simulink model "flightControlSystem"  (R2026a)
settings: Solver=ode3  StartTime=0  StopTime=TFinal  FixedStep=Ts  EnableMultiTasking=on
undefined symbols (not defined in the file): codertarget, Controller, DiscIntNeverNeededParam, Discrete, Estimator, g, init, Sensors, Time, Ts, var_acc_angle_N, var_bias_gyr_N, var_gyro_p_N, Vehicle
libraries: simulink x39, slpidlib x4, ctrlSharedLib x4, sharedtransform x3, parrotlib x1
(part 1 of 2)
settings Model: ExtModeTrigDuration=80  Creator=The MathWorks, Inc.  LastModifiedBy=The MathWorks, Inc.
settings DataIOCC: SaveFormat=StructureWithTime
settings OptimizationCC: PassReuseOutputArgsThreshold=0.0
settings DebuggingCC: ParameterPrecisionLossMsg=none  BusObjectLabelMismatch=error  PregeneratedLibrarySubsystemCodeDiagnostic=none
settings HardwareCC: ProdLargestAtomicInteger=Long  ProdHWDeviceType=ARM Compatible->ARM 9  UseEmbeddedCoderFeatures=off  UseSimulinkCoderFeatures=off
settings ModelReferenceCC: ModelReferenceNumInstancesAllowed=Single
settings RTWCC: SystemTargetFile=ert.tlc  HardwareBoard=PARROT Mambo  TLCOptions=-aInlineSetEventsForThisBaseRateFcn=TLC_FALSE -aSuppressMultiTaskScheduler=TLC_FALSE -aRateBasedStepFcn=1  Toolchain=Sourcery G++ Lite GNU Toolchain for Drones  Description=Embedded Coder
settings CodeAppCC: MaxIdLength=63.0
settings ERTTargetCC: ExtModeMaxTrigDuration=80.0  DynamicArrayContainerType=coder::array  ERTCustomFileBanners=off  MatFileLogging=on  SubcomponentCodeInterfacePackaging=Nonreusable function  SupportContinuousTime=on  SupportNonInlinedSFcns=on  ModelStepFunctionPrototypeControlCompliant=off
settings SimscapeCC: SimscapeLogType=none  SimscapeNominalValues="[{\"value\":\"1\",\"unit\":\"A\"},{\"value\":\"1\",\"unit\":\"bar\"},{\"value\":\"1\",\"unit\":\"cm^2\"},{\"value\":\"1\",\"unit\":\"cm^3/s\"},{\"value\":\"1\",\"unit\":\"kJ/kg\"},{\"value\":\"1\",\"unit\":\"kW\"},{\"value\":\"1\",\"unit\":\"l\"},{\"value\":\"1\",\"unit\":\"N\"},{\"value\":\"1\",\"unit\":\"N*m\"},{\"value\":\"1\",\"unit\":\"V\"}]"  SimscapeLogDataHistory=5000  SimscapeLogDecimation=1

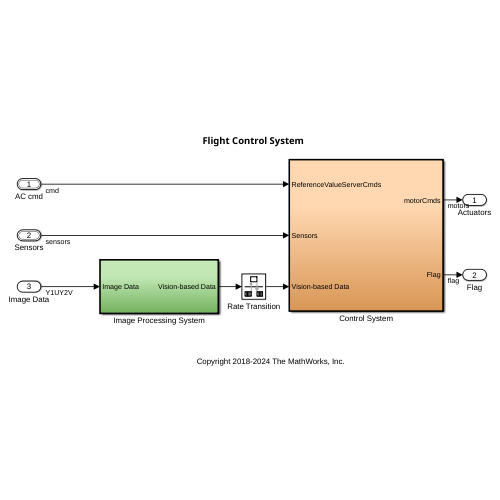
[thumbnail: Simulink's stored preview of the top-level diagram]
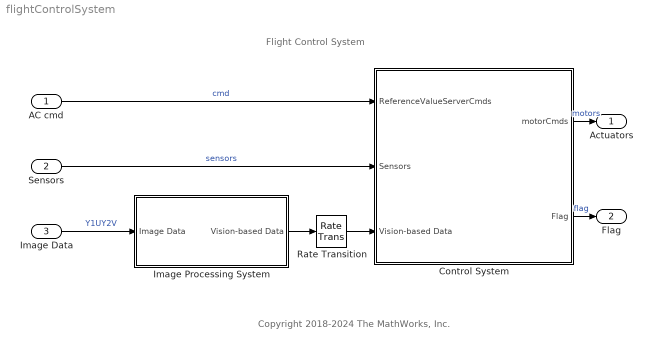
== system flightControlSystem ==
  note: Copyright 2018-2024 The MathWorks, Inc.
  note: Flight Control System
  AC cmd : Inport  OutDataTypeStr=Bus: CommandBus  BusOutputAsStruct=on
  Sensors : Inport  Port=2  OutDataTypeStr=Bus: SensorsBus  BusOutputAsStruct=on
  Image Data : Inport  Tag=IP_IN  InitFcn=codertarget.parrot.internal.inportCallback(gcb);  Port=3  OutDataTypeStr=uint8  PortDimensions=[4 9600]  BusOutputAsStruct=on
  Control System : Subsystem  InitFcn=codertarget.parrot.internal.fcsSubsystemCallback(gcb);  TreatAsAtomicUnit=on  SystemSampleTime=Ts
  Image Processing System : Subsystem  Tag=IP_SUB  InitFcn=codertarget.parrot.internal.ipSubsystemCallback(gcb);  TreatAsAtomicUnit=on  SystemSampleTime=40*Ts  RTWFcnName=ImageFunction
      settings: RTWSystemCode=Inline  RTWFcnNameOpts=User specified
  Rate Transition : RateTransition  Deterministic=off
  Actuators : Outport  OutDataTypeStr=single  PortDimensions=4  VectorParamsAs1DForOutWhenUnconnected=off
  Flag : Outport  Port=2  OutDataTypeStr=uint8  PortDimensions=1  VectorParamsAs1DForOutWhenUnconnected=off
  wires:
  AC cmd/1 -> Control System/1(ReferenceValueServerCmds)  "cmd"
  Control System/1(motorCmds) -> Actuators/1  "motors"
  Sensors/1 -> Control System/2(Sensors)  "sensors"
  Control System/2(Flag) -> Flag/1  "flag"
  Image Data/1 -> Image Processing System/1(Image Data)  "Y1UY2V"
  Image Processing System/1(Vision-based Data) -> Rate Transition/1
  Rate Transition/1 -> Control System/3(Vision-based Data)

== system flightControlSystem/Control System ==
  note: Position or Orientation Control
  note: Use this subsystem to change the path of the
      | Minidrone depending on the input Vision-based
      | Data
  note: Derived from the work by Sertac
      | Karaman and Fabian Riether
  ReferenceValueServerCmds : Inport  OutDataTypeStr=Bus: CommandBus
  Sensors : Inport  Port=2  OutDataTypeStr=Bus: SensorsBus  BusOutputAsStruct=on
  Vision-based Data : Inport  Port=3
  Bus Selector1 : BusSelector  OutputSignals=opticalFlow_data
  Bus Selector4 : BusSelector  OutputSignals=VisionSensors,SensorCalibration
  Control Mode Update : BusAssignment  AssignedSignals=controlModePosVSOrient
  Controller : Subsystem
  Crash Predictor Flags : Subsystem
  Path Planning : Subsystem
  State Estimator : Subsystem
  To Workspace : ToWorkspace  VariableName=estimatedStates  SaveFormat=Structure With Time  SampleTime=-1
  controlModePosVsOrient : Constant  OutDataTypeStr=boolean
  motorCmds : Outport  VectorParamsAs1DForOutWhenUnconnected=off
  Flag : Outport  Port=2  VectorParamsAs1DForOutWhenUnconnected=off
  wires:
  ReferenceValueServerCmds/1 -> Control Mode Update/1
  Bus Selector1/1 -> State Estimator/3(opticalFlow_datin)  "<opticalFlow_data>"
  Bus Selector4/2 -> State Estimator/4(sensorCalibration_datin)  "<SensorCalibration>"
  Path Planning/1(UpdatedReferenceCmds) -> Controller/1(ReferenceValueServerBus)
  Bus Selector4/1 -> Bus Selector1/1  "<VisionSensors>"
  Vision-based Data/1 -> Path Planning/3(Vision-based Data)
  Crash Predictor Flags/1(Flag) -> Flag/1
  Control Mode Update/1 -> Path Planning/1(ReferenceValueServerCmds)
  controlModePosVsOrient/1 -> State Estimator/1(controlModePosVSOrient_flagin), Control Mode Update/2
  Controller/1(motors_refout) -> motorCmds/1
  Sensors/1 -> State Estimator/2(sensor_data_in), Crash Predictor Flags/3(Sensors), Bus Selector4/1
  State Estimator/1(states_estim) -> Controller/2(states_estim), Path Planning/2(EstimatedVal), To Workspace/1, Crash Predictor Flags/1(states_estim)
  State Estimator/2(Alt_prs) -> Crash Predictor Flags/2(Alt_prs)

== system flightControlSystem/Image Processing System ==
  note: Find the dominance of blue in the image
  note: Find the B-(R/2)-(G/2) image
  note: Obtain the RGB image from camera
  Image Data : Inport
  Add : Sum  Inputs=--+
  Constant : Constant  Value=2
  Divide1 : Product  Inputs=/*
  Divide2 : Product  Inputs=*/
  PARROT Image Conversion : parrotlib/PARROT Image Conversion  ImageFormat=RGB  R=on  Y=on  G=on  U=on  B=on  V=on
  RGB Image : VideoViewer  imagePorts=separate color signals  FigPos=[1088 996 418 304]
  Sum of white pixels : Sum  Inputs=+  OutDataTypeStr=uint16
  Threshold for each pixel : simulink/Logic and Bit Operations/Compare To Constant  relop=>  const=50  OutDataTypeStr=boolean
  Threshold for total white pixels : simulink/Logic and Bit Operations/Compare To Constant  relop=>  const=1400  OutDataTypeStr=boolean
  Vision-based Data : Outport  VectorParamsAs1DForOutWhenUnconnected=off
  wires:
  Image Data/1 -> PARROT Image Conversion/1
  Threshold for total white pixels/1 -> Vision-based Data/1
  Add/1 -> Threshold for each pixel/1
  Threshold for each pixel/1 -> Sum of white pixels/1
  Sum of white pixels/1 -> Threshold for total white pixels/1
  Divide2/1 -> Add/1
  PARROT Image Conversion/3 -> RGB Image/3, Add/3
  PARROT Image Conversion/1 -> RGB Image/1, Divide2/1
  PARROT Image Conversion/2 -> RGB Image/2, Divide1/2
  Divide1/1 -> Add/2
  Constant/1 -> Divide1/1, Divide2/2

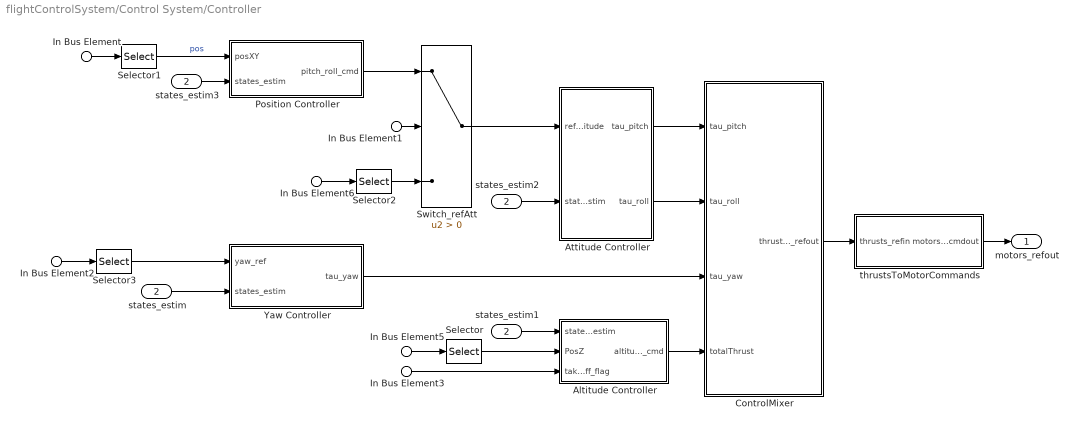
== system flightControlSystem/Control System/Controller ==
  In Bus Element1 : Inport  PortName=ReferenceValueServerBus  Element=controlModePosVSOrient
  In Bus Element : Inport  PortName=ReferenceValueServerBus  Element=pos_ref
  In Bus Element5 : Inport  PortName=ReferenceValueServerBus  Element=pos_ref
  In Bus Element2 : Inport  PortName=ReferenceValueServerBus  Element=orient_ref
  In Bus Element6 : Inport  PortName=ReferenceValueServerBus  Element=orient_ref
  In Bus Element3 : Inport  PortName=ReferenceValueServerBus  Element=takeoff_flag
  states_estim : Inport  Port=2
  Altitude Controller : Subsystem
  Attitude Controller : Subsystem
  ControlMixer : Subsystem
  Position Controller : Subsystem
  Selector : Selector  InputPortWidth=3  IndexOptions=Index vector (dialog)  Indices=3  OutputSizes=1
  Selector1 : Selector  InputPortWidth=3  IndexOptions=Index vector (dialog)  Indices=[1 2]  OutputSizes=1
  Selector2 : Selector  InputPortWidth=3  IndexOptions=Index vector (dialog)  Indices=[2 3]  OutputSizes=1
  Selector3 : Selector  InputPortWidth=3  IndexOptions=Index vector (dialog)  Indices=1  OutputSizes=1
  Switch_refAtt : Switch  Criteria=u2 > Threshold  SaturateOnIntegerOverflow=off  InputSameDT=off
  Yaw Controller : Subsystem
  states_estim1 : InportShadow  Port=2
  states_estim2 : InportShadow  Port=2
  states_estim3 : InportShadow  Port=2
  thrustsToMotorCommands : Subsystem
  motors_refout : Outport  VectorParamsAs1DForOutWhenUnconnected=off
  wires:
  thrustsToMotorCommands/1(motors_cmdout) -> motors_refout/1
  In Bus Element5/1 -> Selector/1
  states_estim3/1 -> Position Controller/2(states_estim)
  In Bus Element6/1 -> Selector2/1
  Selector3/1 -> Yaw Controller/1(yaw_ref)
  In Bus Element/1 -> Selector1/1
  ControlMixer/1(thrusts_refout) -> thrustsToMotorCommands/1(thrusts_refin)
  Selector2/1 -> Switch_refAtt/3
  Altitude Controller/1(altitude_cmd) -> ControlMixer/4(totalThrust)
  Selector1/1 -> Position Controller/1(posXY)  "pos"
  states_estim1/1 -> Altitude Controller/1(states_estim)
  Selector/1 -> Altitude Controller/2(PosZ)
  In Bus Element3/1 -> Altitude Controller/3(takeoff_flag)
  states_estim/1 -> Yaw Controller/2(states_estim)
  Position Controller/1(pitch_roll_cmd) -> Switch_refAtt/1
  In Bus Element2/1 -> Selector3/1
  In Bus Element1/1 -> Switch_refAtt/2
  Switch_refAtt/1 -> Attitude Controller/1(refAttitude)
  states_estim2/1 -> Attitude Controller/2(states_estim)
  Attitude Controller/1(tau_pitch) -> ControlMixer/1(tau_pitch)
  Attitude Controller/2(tau_roll) -> ControlMixer/2(tau_roll)
  Yaw Controller/1(tau_yaw) -> ControlMixer/3(tau_yaw)

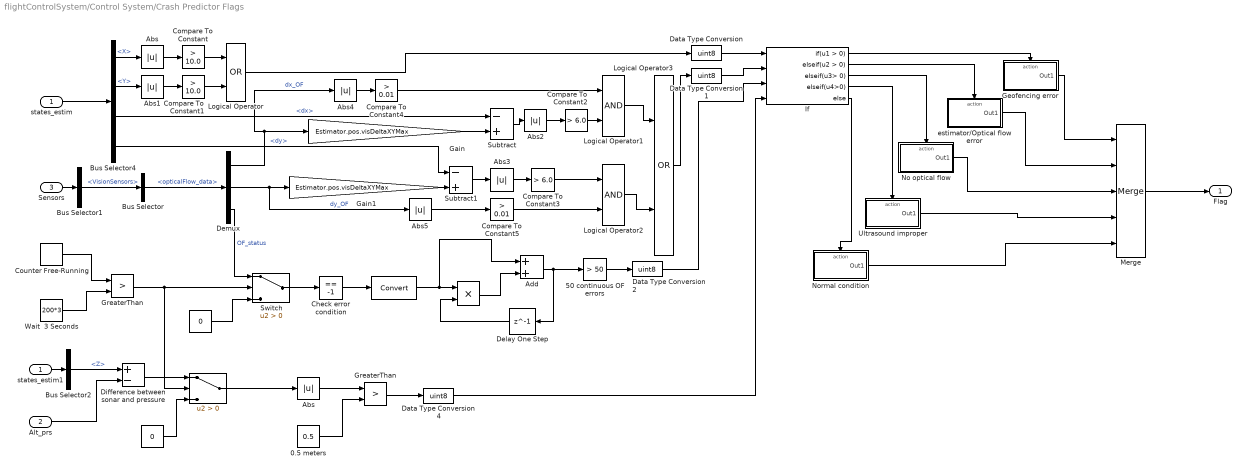
== system flightControlSystem/Control System/Crash Predictor Flags ==
  states_estim : Inport
  Alt_prs : Inport  Port=2
  Sensors : Inport  Port=3
  " " : Constant  Value=0
  "  " : Product  Inputs=**
  "   " : DataTypeConversion  SaturateOnIntegerOverflow=off  RndMeth=Floor
  "    " : Constant  Value=0  OutDataTypeStr=single
  "         " : Switch  Criteria=u2 > Threshold  SaturateOnIntegerOverflow=off  InputSameDT=off
  0.5 meters : Constant  Value=0.5
  "50 continuous OF errors " : simulink/Logic and Bit Operations/Compare To Constant  relop=>  const=50  OutDataTypeStr=boolean
  Abs{,1..5} (6 alike) : Abs  SaturateOnIntegerOverflow=off
  "Abs  " : Abs  SaturateOnIntegerOverflow=off
  Add : Sum
  Bus Selector : BusSelector  OutputSignals=opticalFlow_data
  Bus Selector1 : BusSelector  OutputSignals=VisionSensors
  Bus Selector2 : BusSelector  OutputSignals=Z
  Bus Selector4 : BusSelector  OutputSignals=X,Y,dx,dy
  Check error condition : simulink/Logic and Bit Operations/Compare To Constant  relop===  const=-1  OutDataTypeStr=boolean
  Compare To Constant : simulink/Logic and Bit Operations/Compare To Constant  relop=>  const=10.0  OutDataTypeStr=boolean
  Compare To Constant1 : simulink/Logic and Bit Operations/Compare To Constant  relop=>  const=10.0  OutDataTypeStr=boolean
  Compare To Constant2 : simulink/Logic and Bit Operations/Compare To Constant  relop=>  const=6.0  OutDataTypeStr=boolean
  Compare To Constant3 : simulink/Logic and Bit Operations/Compare To Constant  relop=>  const=6.0  OutDataTypeStr=boolean
  Compare To Constant4 : simulink/Logic and Bit Operations/Compare To Constant  relop=>  const=0.01  OutDataTypeStr=boolean
  Compare To Constant5 : simulink/Logic and Bit Operations/Compare To Constant  relop=>  const=0.01  OutDataTypeStr=boolean
  Counter Free-Running : simulink/Sources/Counter Free-Running  NumBits=32  tsamp=-1
  Data Type Conversion{,1..2,4} (4 alike) : DataTypeConversion  OutDataTypeStr=uint8  RndMeth=Nearest  SaturateOnIntegerOverflow=off
  Delay One Step : Delay  DelayLength=1
  Demux : Demux  Outputs=3
  Difference between sonar and pressure : Sum  Inputs=+-
  Gain : Gain  Gain=Estimator.pos.visDeltaXYMax
  Gain1 : Gain  Gain=Estimator.pos.visDeltaXYMax
  Geofencing error : Subsystem  TreatAsAtomicUnit=on
  GreaterThan : RelationalOperator  Operator=>  OutDataTypeStr=boolean  RndMeth=Simplest  InputSameDT=off
  "GreaterThan  " : RelationalOperator  Operator=>  OutDataTypeStr=boolean  RndMeth=Simplest  InputSameDT=off
  If : If  NumInputs=4  ElseIfExpressions=u2 > 0, u3> 0,u4>0
  Logical Operator : Logic  Operator=OR  AllPortsSameDT=off
  Logical Operator1 : Logic  AllPortsSameDT=off  OutDataTypeStr=boolean
  Logical Operator2 : Logic  AllPortsSameDT=off  OutDataTypeStr=boolean
  Logical Operator3 : Logic  Operator=OR  AllPortsSameDT=off
  Merge : Merge  Inputs=5  InitialOutput=0
  "No optical flow " : Subsystem  TreatAsAtomicUnit=on
  Normal condition : Subsystem  TreatAsAtomicUnit=on
  Subtract : Sum  Inputs=-+
  Subtract1 : Sum  Inputs=-+
  Switch : Switch  Criteria=u2 > Threshold  SaturateOnIntegerOverflow=off  InputSameDT=off
  Ultrasound improper : Subsystem  TreatAsAtomicUnit=on
  Wait  3 Seconds : Constant  Value=200*3
  estimator/Optical flow error : Subsystem  TreatAsAtomicUnit=on
  states_estim1 : InportShadow
  Flag : Outport  VectorParamsAs1DForOutWhenUnconnected=off
  wires:
  Bus Selector4/1 -> Abs/1  "<X>"
  states_estim/1 -> Bus Selector4/1
  Bus Selector4/2 -> Abs1/1  "<Y>"
  Compare To Constant/1 -> Logical Operator/1
  Compare To Constant1/1 -> Logical Operator/2
  Abs/1 -> Compare To Constant/1
  Abs1/1 -> Compare To Constant1/1
  Logical Operator/1 -> Data Type Conversion/1
  Bus Selector/1 -> Demux/1  "<opticalFlow_data>"
  Demux/1 -> Abs4/1, Gain/1  "dx_OF"
  Demux/2 -> Gain1/1, Abs5/1  "dy_OF"
  Bus Selector4/3 -> Subtract/1  "<dx>"
  Subtract/1 -> Abs2/1
  Subtract1/1 -> Abs3/1
  Abs2/1 -> Compare To Constant2/1
  Abs3/1 -> Compare To Constant3/1
  Compare To Constant5/1 -> Logical Operator2/2
  Abs4/1 -> Compare To Constant4/1
  Abs5/1 -> Compare To Constant5/1
  Compare To Constant3/1 -> Logical Operator2/1
  Logical Operator1/1 -> Logical Operator3/1
  Logical Operator2/1 -> Logical Operator3/2
  Logical Operator3/1 -> Data Type Conversion1/1
  Gain/1 -> Subtract/2
  Bus Selector4/4 -> Subtract1/1  "<dy>"
  Gain1/1 -> Subtract1/2
  Compare To Constant4/1 -> Logical Operator1/1
  Compare To Constant2/1 -> Logical Operator1/2
  Sensors/1 -> Bus Selector1/1
  Bus Selector1/1 -> Bus Selector/1  "<VisionSensors>"
  Merge/1 -> Flag/1
  If/1 -> Geofencing error/Action
  If/2 -> estimator/Optical flow error/Action
  If/5 -> Normal condition/Action
  Geofencing error/1(Out1) -> Merge/1
  estimator/Optical flow error/1(Out1) -> Merge/2
  Normal condition/1(Out1) -> Merge/5
  Data Type Conversion/1 -> If/1
  Data Type Conversion1/1 -> If/2
  Check error condition/1 -> "   "/1
  Demux/3 -> Switch/1  "OF_status"
  Delay One Step/1 -> "  "/2
  Add/1 -> Delay One Step/1, "50 continuous OF errors "/1
  "  "/1 -> Add/2
  "50 continuous OF errors "/1 -> Data Type Conversion2/1
  Data Type Conversion2/1 -> If/3
  "No optical flow "/1(Out1) -> Merge/3
  If/3 -> "No optical flow "/Action
  "   "/1 -> Add/1, "  "/1
  Counter Free-Running/1 -> GreaterThan/1
  Wait  3 Seconds/1 -> GreaterThan/2
  Switch/1 -> Check error condition/1
  " "/1 -> Switch/3
  "    "/1 -> "         "/3
  Difference between sonar and pressure/1 -> "         "/1
  Bus Selector2/1 -> Difference between sonar and pressure/1  "<Z>"
  GreaterThan/1 -> Switch/2, "         "/2
  "         "/1 -> "Abs  "/1
  "Abs  "/1 -> "GreaterThan  "/1
  0.5 meters/1 -> "GreaterThan  "/2
  Alt_prs/1 -> Difference between sonar and pressure/2
  "GreaterThan  "/1 -> Data Type Conversion4/1
  states_estim1/1 -> Bus Selector2/1
  Data Type Conversion4/1 -> If/4
  Ultrasound improper/1(Out1) -> Merge/4
  If/4 -> Ultrasound improper/Action

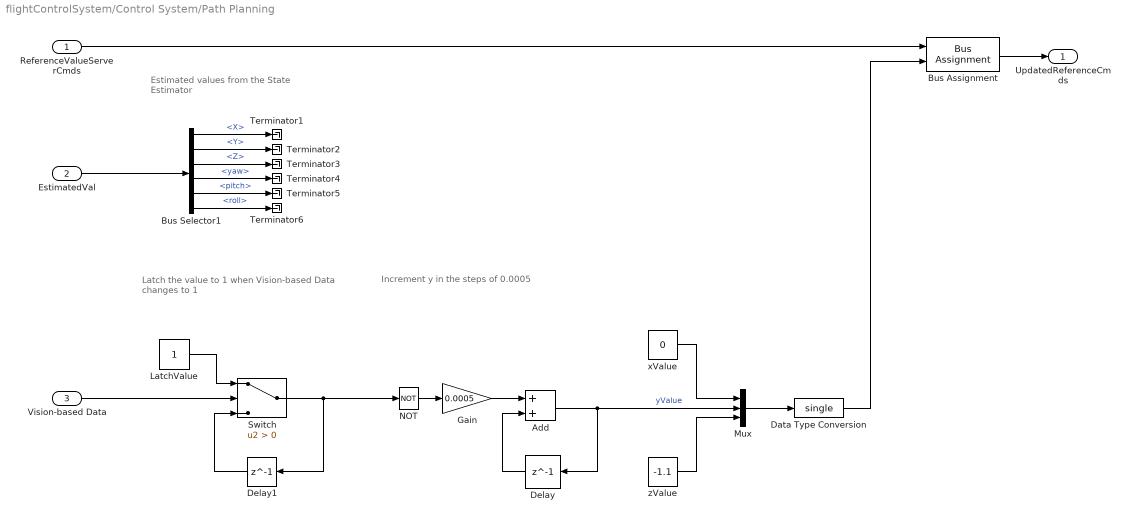
== system flightControlSystem/Control System/Path Planning ==
  note: Increment y in the steps of 0.0005
  note: Latch the value to 1 when
      | Vision-based Data changes to 1
  note: Estimated values from the
      | State Estimator
  ReferenceValueServerCmds : Inport
  EstimatedVal : Inport  Port=2
  Vision-based Data : Inport  Port=3
  Add : Sum
  Bus Selector1 : BusSelector  OutputSignals=X,Y,Z,yaw,pitch,roll
  Bus Assignment : BusAssignment  AssignedSignals=pos_ref
  Data Type Conversion : DataTypeConversion  OutDataTypeStr=single  SaturateOnIntegerOverflow=off  RndMeth=Floor
  Delay : Delay  DelayLength=1
  Delay1 : Delay  DelayLength=1
  Gain : Gain  Gain=0.0005
  LatchValue : Constant
  Mux : Mux  Inputs=3
  NOT : Logic  Operator=NOT  IconShape=distinctive  AllPortsSameDT=off  OutDataTypeStr=boolean
  Switch : Switch  Criteria=u2 > Threshold  SaturateOnIntegerOverflow=off  InputSameDT=off
  Terminator{1..6} (6 alike) : Terminator
  xValue : Constant  Value=0
  zValue : Constant  Value=-1.1
  UpdatedReferenceCmds : Outport  VectorParamsAs1DForOutWhenUnconnected=off
  wires:
  Bus Assignment/1 -> UpdatedReferenceCmds/1
  ReferenceValueServerCmds/1 -> Bus Assignment/1
  Mux/1 -> Data Type Conversion/1
  EstimatedVal/1 -> Bus Selector1/1
  xValue/1 -> Mux/1
  Bus Selector1/1 -> Terminator1/1  "<X>"
  Bus Selector1/2 -> Terminator2/1  "<Y>"
  Bus Selector1/3 -> Terminator3/1  "<Z>"
  Bus Selector1/4 -> Terminator4/1  "<yaw>"
  Bus Selector1/5 -> Terminator5/1  "<pitch>"
  Bus Selector1/6 -> Terminator6/1  "<roll>"
  zValue/1 -> Mux/3
  Data Type Conversion/1 -> Bus Assignment/2
  Delay/1 -> Add/2
  Add/1 -> Delay/1, Mux/2  "yValue"
  Gain/1 -> Add/1
  Vision-based Data/1 -> Switch/2
  LatchValue/1 -> Switch/1
  NOT/1 -> Gain/1
  Switch/1 -> NOT/1, Delay1/1
  Delay1/1 -> Switch/3

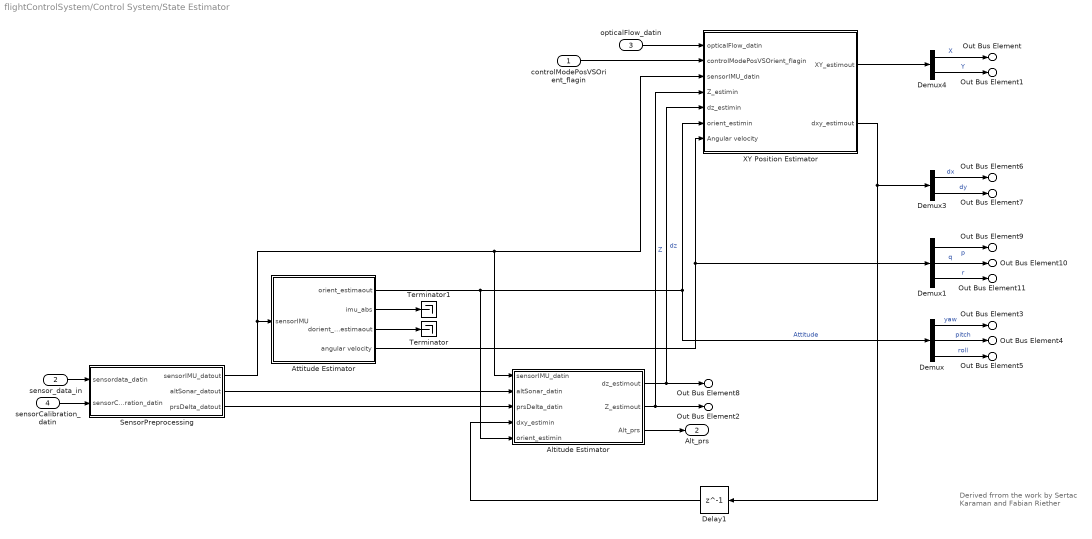
== system flightControlSystem/Control System/State Estimator ==
  note: Derived frrom the work by Sertac
      | Karaman and Fabian Riether
  controlModePosVSOrient_flagin : Inport  OutDataTypeStr=boolean
  sensor_data_in : Inport  Port=2
  opticalFlow_datin : Inport  Port=3
  sensorCalibration_datin : Inport  Port=4
  Altitude Estimator : Subsystem
  Attitude Estimator : Subsystem
  Delay1 : Delay  DelayLength=1  InitialCondition=0
  Demux : Demux  Outputs=3
  Demux1 : Demux  Outputs=3
  Demux3 : Demux  Outputs=2
  Demux4 : Demux  Outputs=2
  SensorPreprocessing : Subsystem
  Terminator : Terminator
  Terminator1 : Terminator
  XY Position Estimator : Subsystem
  Out Bus Element : Outport  VectorParamsAs1DForOutWhenUnconnected=off  PortName=states_estim  Element=X
  Out Bus Element1 : Outport  VectorParamsAs1DForOutWhenUnconnected=off  PortName=states_estim  Element=Y
  Out Bus Element2 : Outport  VectorParamsAs1DForOutWhenUnconnected=off  PortName=states_estim  Element=Z
  Out Bus Element3 : Outport  VectorParamsAs1DForOutWhenUnconnected=off  PortName=states_estim  Element=yaw
  Out Bus Element4 : Outport  VectorParamsAs1DForOutWhenUnconnected=off  PortName=states_estim  Element=pitch
  Out Bus Element5 : Outport  VectorParamsAs1DForOutWhenUnconnected=off  PortName=states_estim  Element=roll
  Out Bus Element6 : Outport  VectorParamsAs1DForOutWhenUnconnected=off  PortName=states_estim  Element=dx
  Out Bus Element7 : Outport  VectorParamsAs1DForOutWhenUnconnected=off  PortName=states_estim  Element=dy
  Out Bus Element8 : Outport  VectorParamsAs1DForOutWhenUnconnected=off  PortName=states_estim  Element=dz
  Out Bus Element9 : Outport  VectorParamsAs1DForOutWhenUnconnected=off  PortName=states_estim  Element=p
  Out Bus Element10 : Outport  VectorParamsAs1DForOutWhenUnconnected=off  PortName=states_estim  Element=q
  Out Bus Element11 : Outport  VectorParamsAs1DForOutWhenUnconnected=off  PortName=states_estim  Element=r
  Alt_prs : Outport  Port=2  VectorParamsAs1DForOutWhenUnconnected=off
  wires:
  XY Position Estimator/2(dxy_estimout) -> Demux3/1, Delay1/1
  Demux1/3 -> Out Bus Element11/1  "r"
  Demux/3 -> Out Bus Element5/1  "roll"
  Demux4/2 -> Out Bus Element1/1  "Y"
  XY Position Estimator/1(XY_estimout) -> Demux4/1
  Attitude Estimator/2(imu_abs) -> Terminator1/1
  Attitude Estimator/4(angular velocity) -> XY Position Estimator/7(Angular velocity), Demux1/1
  sensor_data_in/1 -> SensorPreprocessing/1(sensordata_datin)
  opticalFlow_datin/1 -> XY Position Estimator/1(opticalFlow_datin)
  Demux4/1 -> Out Bus Element/1  "X"
  SensorPreprocessing/1(sensorIMU_datout) -> Attitude Estimator/1(sensorIMU), XY Position Estimator/3(sensorIMU_datin), Altitude Estimator/1(sensorIMU_datin)
  SensorPreprocessing/3(prsDelta_datout) -> Altitude Estimator/3(prsDelta_datin)
  Demux3/2 -> Out Bus Element7/1  "dy"
  SensorPreprocessing/2(altSonar_datout) -> Altitude Estimator/2(altSonar_datin)
  Altitude Estimator/1(dz_estimout) -> XY Position Estimator/5(dz_estimin), Out Bus Element8/1  "dz"
  Altitude Estimator/2(Z_estimout) -> XY Position Estimator/4(Z_estimin), Out Bus Element2/1  "Z"
  Demux1/1 -> Out Bus Element9/1  "p"
  Demux3/1 -> Out Bus Element6/1  "dx"
  Attitude Estimator/3(dorient_estimaout) -> Terminator/1
  Demux/2 -> Out Bus Element4/1  "pitch"
  controlModePosVSOrient_flagin/1 -> XY Position Estimator/2(controlModePosVSOrient_flagin)
  Attitude Estimator/1(orient_estimaout) -> XY Position Estimator/6(orient_estimin), Demux/1, Altitude Estimator/5(orient_estimin)  "Attitude"
  Demux/1 -> Out Bus Element3/1  "yaw"
  Delay1/1 -> Altitude Estimator/4(dxy_estimin)
  Demux1/2 -> Out Bus Element10/1  "q"
  sensorCalibration_datin/1 -> SensorPreprocessing/2(sensorCalibration_datin)
  Altitude Estimator/3(Alt_prs) -> Alt_prs/1

== system flightControlSystem/Control System/Controller/Altitude Controller ==
  note: PID Controller for Altitude
  note: ALTITUDE CONTROLLER
  states_estim : Inport
  PosZ : Inport  Port=2
  takeoff_flag : Inport  Port=3
  Bus Selector1 : BusSelector  OutputSignals=Z,dz
  Compare To Constant : simulink/Logic and Bit Operations/Compare To Constant  relop=<  const=100  OutDataTypeStr=boolean
  Counter Free-Running : simulink/Sources/Counter Free-Running  NumBits=16  tsamp=-1
  D_z1 : Gain  Gain=0.5  ParamDataTypeStr=single  OutDataTypeStr=single  SaturateOnIntegerOverflow=on
  Discrete-Time Integrator : DiscreteIntegrator  ExternalReset=falling  SampleTime=Ts  LimitOutput=on  UpperSaturationLimit=2  LowerSaturationLimit=-2  ICPrevOutput=DiscIntNeverNeededParam  ICPrevScaledInput=DiscIntNeverNeededParam
  I_pr : Gain  Gain=0.24
  P_z1 : Gain  Gain=0.8  ParamDataTypeStr=single  OutDataTypeStr=single  SaturateOnIntegerOverflow=on
  SaturationThrust1 : Saturate  UpperLimit=4*Controller.totalThrustMaxRelative*Controller.motorsThrustPerMotorMax  LowerLimit=-4*Controller.totalThrustMaxRelative*Controller.motorsThrustPerMotorMax  OutDataTypeStr=single
  Sum1 : Sum  Inputs=++-  OutDataTypeStr=single  AccumDataTypeStr=single  SaturateOnIntegerOverflow=on
  Sum2 : Sum  Inputs=+-|  OutDataTypeStr=single  AccumDataTypeStr=single  SaturateOnIntegerOverflow=on
  Sum5 : Sum  Inputs=++|  OutDataTypeStr=single  AccumDataTypeStr=single  SaturateOnIntegerOverflow=on
  TakeoffOrControl_Switch1 : Switch  Criteria=u2 > Threshold  SaturateOnIntegerOverflow=off  InputSameDT=off
  Terminator : Terminator
  takeoff_gain1 : Gain  Gain=Controller.takeoffGain  ParamDataTypeStr=single  OutDataTypeStr=single  SaturateOnIntegerOverflow=on
  w1 : Constant  Value=-g*Vehicle.Airframe.mass  OutDataTypeStr=single  SampleTime=Ts
  altitude_cmd : Outport  VectorParamsAs1DForOutWhenUnconnected=off
  wires:
  TakeoffOrControl_Switch1/1 -> Sum5/2
  Discrete-Time Integrator/1 -> Sum1/1
  PosZ/1 -> Sum2/1
  takeoff_flag/1 -> Terminator/1
  w1/1 -> Sum5/1, takeoff_gain1/1  "Feed forward term to  compensate for gravity"
  P_z1/1 -> Sum1/2
  Counter Free-Running/1 -> Compare To Constant/1
  Bus Selector1/2 -> D_z1/1  "<dz>"
  Sum5/1 -> SaturationThrust1/1
  Bus Selector1/1 -> Sum2/2  "<Z>"
  D_z1/1 -> Sum1/3  "dz"
  Sum1/1 -> TakeoffOrControl_Switch1/3
  Compare To Constant/1 -> Discrete-Time Integrator/2, TakeoffOrControl_Switch1/2
  takeoff_gain1/1 -> TakeoffOrControl_Switch1/1
  states_estim/1 -> Bus Selector1/1
  Sum2/1 -> I_pr/1, P_z1/1  "pitch/roll error"
  I_pr/1 -> Discrete-Time Integrator/1
  SaturationThrust1/1 -> altitude_cmd/1

== system flightControlSystem/Control System/Controller/Attitude Controller ==
  note: Inner loop PID
      | controls angular velocity
  note: Outer Proportional loop
      | controls the pitch and roll angle
  note: ATTITUDE CONTROL
  refAttitude : Inport
  states_estim : Inport  Port=2
  Angle control loop : slpidlib/PID Controller  Controller=P  Form=Parallel  TimeDomain=Discrete-time  UseExternalTs=off  SampleTime=Ts  IntegratorMethod=Forward Euler  FilterMethod=Forward Euler  ControllerParametersSource=internal  P=4  I=1  UseKiTs=off  D=0  UseExternalDerivativeSource=off  N=100  UseFilter=on  TunerSelectOption=Transfer Function Based (PID Tuner App)  InitialConditionSource=internal  InitialConditionForIntegrator=0  InitialConditionForFilter=0  DifferentiatorICPrevScaledInput=0  ExternalReset=none  TrackingMode=off  Kt=1  LimitOutput=off  SatLimitsSource=internal  UpperSaturationLimit=inf  LowerSaturationLimit=-inf  LinearizeAsGain=on  AntiWindupMode=none  Kb=1  LimitIntegrator=off  UpperIntegratorSaturationLimit=inf  LowerIntegratorSaturationLimit=-inf  POutMin=[]  POutMax=[]  IOutMin=[]  IOutMax=[]  DOutMin=[]  DOutMax=[]  NOutMin=[]  NOutMax=[]  SumOutMin=[]  SumOutMax=[]  SaturationOutMin=[]  SaturationOutMax=[]  PParamMin=[]  PParamMax=[]  IParamMin=[]  IParamMax=[]  DParamMin=[]  DParamMax=[]  NParamMin=[]  NParamMax=[]  KbParamMin=[]  KbParamMax=[]  KtParamMin=[]  KtParamMax=[]  KbOutMin=[]  KbOutMax=[]  KtOutMin=[]  KtOutMax=[]  IntegratorOutMin=[]  IntegratorOutMax=[]  FilterOutMin=[]  FilterOutMax=[]  SumI1OutMin=[]  SumI1OutMax=[]  SumI2OutMin=[]  SumI2OutMax=[]  SumI3OutMin=[]  SumI3OutMax=[]  SumI4OutMin=[]  SumI4OutMax=[]  SumDOutMin=[]  SumDOutMax=[]  DifferentiatorOutMin=[]  DifferentiatorOutMax=[]  FilterDiffOutCoefMin=[]  FilterDiffOutCoefMax=[]  ReciprocalOutMin=[]  ReciprocalOutMax=[]  SumDenOutMin=[]  SumDenOutMax=[]  SumNumOutMin=[]  SumNumOutMax=[]  DivideOutMin=[]  DivideOutMax=[]  UdiffTsProdOutMin=[]  UdiffTsProdOutMax=[]  NTsProdOutMin=[]  NTsProdOutMax=[]  UintegralTsProdOutMin=[]  UintegralTsProdOutMax=[]  UngainTsProdOutMin=[]  UngainTsProdOutMax=[]  ClampingZeroOutDataTypeStr=Inherit: Inherit via back propagation  ClampingZeroOutMin=[]  ClampingZeroOutMax=[]  FilterDenConstantOutDataTypeStr=Inherit: Inherit via back propagation  FilterDenConstantOutMin=[]  FilterDenConstantOutMax=[]  PCopyOutDataTypeStr=Inherit: Inherit via back propagation  PCopyOutMin=[]  PCopyOutMax=[]  NCopyOutDataTypeStr=Inherit: Inherit via back propagation  NCopyOutMin=[]  NCopyOutMax=[]  IntegratorContinuousStateAttributes=''  IntegratorStateMustResolveToSignalObject=off  IntegratorRTWStateStorageClass=Auto  FilterContinuousStateAttributes=''  FilterStateMustResolveToSignalObject=off  FilterRTWStateStorageClass=Auto  ParallelPVariant=InternalParameters  IdealPVariant=Disabled  IVariant=Disabled  DVariant=Disabled  IntegratorVariant=Disabled  SatVariant=Disabled  AWVariant=Disabled  PCopyVariant=Disabled  TRVariant=Disabled  FdbkBlocksVariant=Forward  IdealPFdbkVariant=Disabled  SatFdbkVariant=Disabled  DerivativeFilterVariant=Disabled  NVariant=Disabled  NCopyVariant=Disabled_SignalSpec  FilterICVariant=Disabled  IntegratorICVariant=Disabled  ExternalResetVariant=Disabled  TRSumVariant=Passthrough  SumFdbkVariant=Disabled  SumVariant=Passthrough_P  TsampFilterVariant=InternalTs  TsampNgainVariant=Passthrough  TsampIntegralVariant=Disabled_SignalSpec  ExternalSaturationOutDataTypeStr=Inherit: Same as second input  DerivativeSourceVariant=Disabled  PreIntVariant=InternalPreInt
  Angular velocity control loop : slpidlib/PID Controller  Controller=PID  Form=Parallel  TimeDomain=Discrete-time  UseExternalTs=off  SampleTime=Ts  IntegratorMethod=Forward Euler  FilterMethod=Forward Euler  ControllerParametersSource=internal  P=0.003*[1 0.81]  I=2*0.003*[1 0.81]  UseKiTs=off  D=0.003/25*[1 0.81]  UseExternalDerivativeSource=off  N=70*[1 1]  UseFilter=on  TunerSelectOption=Transfer Function Based (PID Tuner App)  InitialConditionSource=internal  InitialConditionForIntegrator=0  InitialConditionForFilter=0  DifferentiatorICPrevScaledInput=0  ExternalReset=none  TrackingMode=off  Kt=1  LimitOutput=on  SatLimitsSource=internal  UpperSaturationLimit=0.02  LowerSaturationLimit=-0.02  LinearizeAsGain=on  AntiWindupMode=clamping  Kb=1  LimitIntegrator=off  UpperIntegratorSaturationLimit=inf  LowerIntegratorSaturationLimit=-inf  POutMin=[]  POutMax=[]  IOutMin=[]  IOutMax=[]  DOutMin=[]  DOutMax=[]  NOutMin=[]  NOutMax=[]  SumOutMin=[]  SumOutMax=[]  SaturationOutMin=[]  SaturationOutMax=[]  PParamMin=[]  PParamMax=[]  IParamMin=[]  IParamMax=[]  DParamMin=[]  DParamMax=[]  NParamMin=[]  NParamMax=[]  KbParamMin=[]  KbParamMax=[]  KtParamMin=[]  KtParamMax=[]  KbOutMin=[]  KbOutMax=[]  KtOutMin=[]  KtOutMax=[]  IntegratorOutMin=[]  IntegratorOutMax=[]  FilterOutMin=[]  FilterOutMax=[]  SumI1OutMin=[]  SumI1OutMax=[]  SumI2OutMin=[]  SumI2OutMax=[]  SumI3OutMin=[]  SumI3OutMax=[]  SumI4OutMin=[]  SumI4OutMax=[]  SumDOutMin=[]  SumDOutMax=[]  DifferentiatorOutMin=[]  DifferentiatorOutMax=[]  FilterDiffOutCoefMin=[]  FilterDiffOutCoefMax=[]  ReciprocalOutMin=[]  ReciprocalOutMax=[]  SumDenOutMin=[]  SumDenOutMax=[]  SumNumOutMin=[]  SumNumOutMax=[]  DivideOutMin=[]  DivideOutMax=[]  UdiffTsProdOutMin=[]  UdiffTsProdOutMax=[]  NTsProdOutMin=[]  NTsProdOutMax=[]  UintegralTsProdOutMin=[]  UintegralTsProdOutMax=[]  UngainTsProdOutMin=[]  UngainTsProdOutMax=[]  ClampingZeroOutDataTypeStr=Inherit: Inherit via back propagation  ClampingZeroOutMin=[]  ClampingZeroOutMax=[]  FilterDenConstantOutDataTypeStr=Inherit: Inherit via back propagation  FilterDenConstantOutMin=[]  FilterDenConstantOutMax=[]  PCopyOutDataTypeStr=Inherit: Inherit via back propagation  PCopyOutMin=[]  PCopyOutMax=[]  NCopyOutDataTypeStr=Inherit: Inherit via back propagation  NCopyOutMin=[]  NCopyOutMax=[]  IntegratorContinuousStateAttributes=''  IntegratorStateMustResolveToSignalObject=off  IntegratorRTWStateStorageClass=Auto  FilterContinuousStateAttributes=''  FilterStateMustResolveToSignalObject=off  FilterRTWStateStorageClass=Auto  ParallelPVariant=InternalParameters  IdealPVariant=Disabled  IVariant=InternalParameters  DVariant=InternalParameters  IntegratorVariant=Discrete  SatVariant=Enabled  AWVariant=DiscClampingParallel  PCopyVariant=Disabled  TRVariant=Disabled  FdbkBlocksVariant=Forward  IdealPFdbkVariant=Disabled  SatFdbkVariant=Disabled  DerivativeFilterVariant=ForwardEulerFilter  NVariant=InternalParameters  NCopyVariant=Disabled  FilterICVariant=InternalICsFilter  IntegratorICVariant=InternalICs  ExternalResetVariant=Disabled  TRSumVariant=Passthrough  SumFdbkVariant=Disabled  SumVariant=Sum_PID  TsampFilterVariant=InternalTs  TsampNgainVariant=Passthrough  TsampIntegralVariant=Disabled_SignalSpec  ExternalSaturationOutDataTypeStr=Inherit: Same as second input  DerivativeSourceVariant=ErrorSignal  PreIntVariant=InternalPreInt
  Bus Selector1 : BusSelector  OutputSignals=q,p
  Bus Selector3 : BusSelector  OutputSignals=pitch,roll
  Demux1 : Demux  Outputs=2
  Mux : Mux  Inputs=2
  Mux2 : Mux  Inputs=2
  Sum1 : Sum  Inputs=|+-
  Sum19 : Sum  Inputs=|+-
  tau_pitch : Outport  VectorParamsAs1DForOutWhenUnconnected=off
  tau_roll : Outport  Port=2  VectorParamsAs1DForOutWhenUnconnected=off
  wires:
  Sum1/1 -> Angular velocity control loop/1  "pitch/roll error"
  Angle control loop/1 -> Sum1/1
  Mux2/1 -> Sum1/2
  Sum19/1 -> Angle control loop/1  "pitch/roll error"
  Angular velocity control loop/1 -> Demux1/1
  Demux1/2 -> tau_roll/1  "tau_roll"
  Demux1/1 -> tau_pitch/1  "tau_pitch"
  Bus Selector3/2 -> Mux/2  "<roll>"
  Mux/1 -> Sum19/2
  refAttitude/1 -> Sum19/1
  states_estim/1 -> Bus Selector1/1, Bus Selector3/1
  Bus Selector3/1 -> Mux/1  "<pitch>"
  Bus Selector1/1 -> Mux2/1  "<q>"
  Bus Selector1/2 -> Mux2/2  "<p>"

== system flightControlSystem/Control System/Controller/ControlMixer ==
  tau_pitch : Inport
  tau_roll : Inport  Port=2
  tau_yaw : Inport  Port=3
  totalThrust : Inport  Port=4
  Add : Sum
  Manual Switch : ManualSwitch
  Mux2 : Mux
  Pitch correction : Constant  Value=0.002  OutDataTypeStr=single
  Product : Product  Multiplication=Matrix(*)  RndMeth=Zero
  TorqueTotalThrustToThrustPerMotor : Constant  Value=Controller.Q2Ts  OutDataTypeStr=single
  Variant Source : VariantSource  VariantControlMode=sim codegen switching  VariantActivationTime=update diagram analyze all choices  ShowConditionOnBlock=on  VariantControls={(sim), (codegen)}
  zero correction : Constant  Value=0  OutDataTypeStr=single
  thrusts_refout : Outport  VectorParamsAs1DForOutWhenUnconnected=off
  wires:
  Product/1 -> thrusts_refout/1
  tau_roll/1 -> Mux2/4
  Add/1 -> Variant Source/2
  tau_yaw/1 -> Mux2/2
  totalThrust/1 -> Mux2/1
  TorqueTotalThrustToThrustPerMotor/1 -> Product/1
  Mux2/1 -> Product/2
  Variant Source/1 -> Mux2/3
  tau_pitch/1 -> Add/1, Variant Source/1
  Pitch correction/1 -> Manual Switch/1
  zero correction/1 -> Manual Switch/2
  Manual Switch/1 -> Add/2

== system flightControlSystem/Control System/Controller/Position Controller ==
  note: Position controller requires good estimate of Yaw orientation to work properly.
      | Incase position control is not needed, the outer loop can be removed and velocity setpoint can be given directly
  note: Inner loop controls linear velocity error
  note: Outer loop controls the position error
  posXY : Inport
  states_estim : Inport  Port=2
  Bus Selector1 : BusSelector  OutputSignals=X,Y
  Bus Selector2 : BusSelector  OutputSignals=dx,dy
  Bus Selector3 : BusSelector  OutputSignals=yaw
  Gain : Gain  Gain=[-1, 1]
  LPF 8Hz Cutoff Filter to avoid oscillations induced by position controller : DiscreteTransferFcn  Numerator=[1, 1]  Denominator=[1+1/pi/Ts/8, 1-1/pi/Ts/8]
  Mux : Mux  Inputs=2
  Mux1 : Mux  Inputs=2
  Position controller : slpidlib/PID Controller  Controller=P  Form=Parallel  TimeDomain=Discrete-time  UseExternalTs=off  SampleTime=Ts  IntegratorMethod=Forward Euler  FilterMethod=Forward Euler  ControllerParametersSource=internal  P=0.7  I=0.1  UseKiTs=off  D=0  UseExternalDerivativeSource=off  N=100  UseFilter=on  TunerSelectOption=Transfer Function Based (PID Tuner App)  InitialConditionSource=internal  InitialConditionForIntegrator=0  InitialConditionForFilter=0  DifferentiatorICPrevScaledInput=0  ExternalReset=none  TrackingMode=off  Kt=1  LimitOutput=on  SatLimitsSource=internal  UpperSaturationLimit=0.5  LowerSaturationLimit=-0.5  LinearizeAsGain=on  AntiWindupMode=clamping  Kb=1  LimitIntegrator=off  UpperIntegratorSaturationLimit=inf  LowerIntegratorSaturationLimit=-inf  POutMin=[]  POutMax=[]  IOutMin=[]  IOutMax=[]  DOutMin=[]  DOutMax=[]  NOutMin=[]  NOutMax=[]  SumOutMin=[]  SumOutMax=[]  SaturationOutMin=[]  SaturationOutMax=[]  PParamMin=[]  PParamMax=[]  IParamMin=[]  IParamMax=[]  DParamMin=[]  DParamMax=[]  NParamMin=[]  NParamMax=[]  KbParamMin=[]  KbParamMax=[]  KtParamMin=[]  KtParamMax=[]  KbOutMin=[]  KbOutMax=[]  KtOutMin=[]  KtOutMax=[]  IntegratorOutMin=[]  IntegratorOutMax=[]  FilterOutMin=[]  FilterOutMax=[]  SumI1OutMin=[]  SumI1OutMax=[]  SumI2OutMin=[]  SumI2OutMax=[]  SumI3OutMin=[]  SumI3OutMax=[]  SumI4OutMin=[]  SumI4OutMax=[]  SumDOutMin=[]  SumDOutMax=[]  DifferentiatorOutMin=[]  DifferentiatorOutMax=[]  FilterDiffOutCoefMin=[]  FilterDiffOutCoefMax=[]  ReciprocalOutMin=[]  ReciprocalOutMax=[]  SumDenOutMin=[]  SumDenOutMax=[]  SumNumOutMin=[]  SumNumOutMax=[]  DivideOutMin=[]  DivideOutMax=[]  UdiffTsProdOutMin=[]  UdiffTsProdOutMax=[]  NTsProdOutMin=[]  NTsProdOutMax=[]  UintegralTsProdOutMin=[]  UintegralTsProdOutMax=[]  UngainTsProdOutMin=[]  UngainTsProdOutMax=[]  ClampingZeroOutDataTypeStr=Inherit: Inherit via back propagation  ClampingZeroOutMin=[]  ClampingZeroOutMax=[]  FilterDenConstantOutDataTypeStr=Inherit: Inherit via back propagation  FilterDenConstantOutMin=[]  FilterDenConstantOutMax=[]  PCopyOutDataTypeStr=Inherit: Inherit via back propagation  PCopyOutMin=[]  PCopyOutMax=[]  NCopyOutDataTypeStr=Inherit: Inherit via back propagation  NCopyOutMin=[]  NCopyOutMax=[]  IntegratorContinuousStateAttributes=''  IntegratorStateMustResolveToSignalObject=off  IntegratorRTWStateStorageClass=Auto  FilterContinuousStateAttributes=''  FilterStateMustResolveToSignalObject=off  FilterRTWStateStorageClass=Auto  ParallelPVariant=InternalParameters  IdealPVariant=Disabled  IVariant=Disabled  DVariant=Disabled  IntegratorVariant=Disabled  SatVariant=Enabled  AWVariant=Disabled  PCopyVariant=Disabled  TRVariant=Disabled  FdbkBlocksVariant=Forward  IdealPFdbkVariant=Disabled  SatFdbkVariant=Disabled  DerivativeFilterVariant=Disabled  NVariant=Disabled  NCopyVariant=Disabled_SignalSpec  FilterICVariant=Disabled  IntegratorICVariant=Disabled  ExternalResetVariant=Disabled  TRSumVariant=Passthrough  SumFdbkVariant=Disabled  SumVariant=Passthrough_P  TsampFilterVariant=InternalTs  TsampNgainVariant=Passthrough  TsampIntegralVariant=Disabled_SignalSpec  ExternalSaturationOutDataTypeStr=Inherit: Same as second input  DerivativeSourceVariant=Disabled  PreIntVariant=InternalPreInt
  Position error transformation (Earth to Body frame) : MATLAB Function  TreatAsAtomicUnit=on
  Sum1 : Sum  Inputs=|+-
  Sum19 : Sum  Inputs=|+-
  Velocity controller : slpidlib/PID Controller  Controller=PI  Form=Parallel  TimeDomain=Discrete-time  UseExternalTs=off  SampleTime=Ts  IntegratorMethod=Forward Euler  FilterMethod=Forward Euler  ControllerParametersSource=internal  P=0.2  I=0.1  UseKiTs=off  D=0  UseExternalDerivativeSource=off  N=100  UseFilter=on  TunerSelectOption=Transfer Function Based (PID Tuner App)  InitialConditionSource=internal  InitialConditionForIntegrator=0  InitialConditionForFilter=0  DifferentiatorICPrevScaledInput=0  ExternalReset=none  TrackingMode=off  Kt=1  LimitOutput=on  SatLimitsSource=internal  UpperSaturationLimit=20*pi/180  LowerSaturationLimit=-20*pi/180  LinearizeAsGain=on  AntiWindupMode=clamping  Kb=1  LimitIntegrator=off  UpperIntegratorSaturationLimit=inf  LowerIntegratorSaturationLimit=-inf  POutMin=[]  POutMax=[]  IOutMin=[]  IOutMax=[]  DOutMin=[]  DOutMax=[]  NOutMin=[]  NOutMax=[]  SumOutMin=[]  SumOutMax=[]  SaturationOutMin=[]  SaturationOutMax=[]  PParamMin=[]  PParamMax=[]  IParamMin=[]  IParamMax=[]  DParamMin=[]  DParamMax=[]  NParamMin=[]  NParamMax=[]  KbParamMin=[]  KbParamMax=[]  KtParamMin=[]  KtParamMax=[]  KbOutMin=[]  KbOutMax=[]  KtOutMin=[]  KtOutMax=[]  IntegratorOutMin=[]  IntegratorOutMax=[]  FilterOutMin=[]  FilterOutMax=[]  SumI1OutMin=[]  SumI1OutMax=[]  SumI2OutMin=[]  SumI2OutMax=[]  SumI3OutMin=[]  SumI3OutMax=[]  SumI4OutMin=[]  SumI4OutMax=[]  SumDOutMin=[]  SumDOutMax=[]  DifferentiatorOutMin=[]  DifferentiatorOutMax=[]  FilterDiffOutCoefMin=[]  FilterDiffOutCoefMax=[]  ReciprocalOutMin=[]  ReciprocalOutMax=[]  SumDenOutMin=[]  SumDenOutMax=[]  SumNumOutMin=[]  SumNumOutMax=[]  DivideOutMin=[]  DivideOutMax=[]  UdiffTsProdOutMin=[]  UdiffTsProdOutMax=[]  NTsProdOutMin=[]  NTsProdOutMax=[]  UintegralTsProdOutMin=[]  UintegralTsProdOutMax=[]  UngainTsProdOutMin=[]  UngainTsProdOutMax=[]  ClampingZeroOutDataTypeStr=Inherit: Inherit via back propagation  ClampingZeroOutMin=[]  ClampingZeroOutMax=[]  FilterDenConstantOutDataTypeStr=Inherit: Inherit via back propagation  FilterDenConstantOutMin=[]  FilterDenConstantOutMax=[]  PCopyOutDataTypeStr=Inherit: Inherit via back propagation  PCopyOutMin=[]  PCopyOutMax=[]  NCopyOutDataTypeStr=Inherit: Inherit via back propagation  NCopyOutMin=[]  NCopyOutMax=[]  IntegratorContinuousStateAttributes=''  IntegratorStateMustResolveToSignalObject=off  IntegratorRTWStateStorageClass=Auto  FilterContinuousStateAttributes=''  FilterStateMustResolveToSignalObject=off  FilterRTWStateStorageClass=Auto  ParallelPVariant=InternalParameters  IdealPVariant=Disabled  IVariant=InternalParameters  DVariant=Disabled  IntegratorVariant=Discrete  SatVariant=Enabled  AWVariant=DiscClampingParallel  PCopyVariant=Disabled  TRVariant=Disabled  FdbkBlocksVariant=Forward  IdealPFdbkVariant=Disabled  SatFdbkVariant=Disabled  DerivativeFilterVariant=Disabled  NVariant=Disabled  NCopyVariant=Disabled_SignalSpec  FilterICVariant=Disabled  IntegratorICVariant=InternalICs  ExternalResetVariant=Disabled  TRSumVariant=Passthrough  SumFdbkVariant=Disabled  SumVariant=Sum_PI  TsampFilterVariant=InternalTs  TsampNgainVariant=Passthrough  TsampIntegralVariant=Disabled_SignalSpec  ExternalSaturationOutDataTypeStr=Inherit: Same as second input  DerivativeSourceVariant=Disabled  PreIntVariant=InternalPreInt
  pitch_roll_cmd : Outport  VectorParamsAs1DForOutWhenUnconnected=off
  wires:
  Bus Selector2/1 -> Mux1/1  "<dx>"
  states_estim/1 -> Bus Selector2/1, Bus Selector3/1, Bus Selector1/1
  Bus Selector1/1 -> Mux/1  "<X>"
  Bus Selector1/2 -> Mux/2  "<Y>"
  Bus Selector2/2 -> Mux1/2  "<dy>"
  Mux1/1 -> Sum19/2
  Sum19/1 -> Velocity controller/1
  Velocity controller/1 -> LPF 8Hz Cutoff Filter to avoid oscillations induced by position controller/1
  Gain/1 -> pitch_roll_cmd/1  "Pitch,Roll setpoint"
  LPF 8Hz Cutoff Filter to avoid oscillations induced by position controller/1 -> Gain/1
  Position controller/1 -> Sum19/1  "Velocity  setpoint"
  Mux/1 -> Sum1/2
  Sum1/1 -> Position error transformation (Earth to Body frame)/2(xy_err_earth)
  Position error transformation (Earth to Body frame)/1(xy_err_body) -> Position controller/1
  posXY/1 -> Sum1/1  "Position setpoint"
  Bus Selector3/1 -> Position error transformation (Earth to Body frame)/1(yaw)  "<yaw>"

== system flightControlSystem/Control System/Controller/Yaw Controller ==
  note: Yaw angle is not constrained between -180 to 180 degrees
  note: Yaw estimation is done solely using the gyroscope and it may drift with time.
  yaw_ref : Inport
  states_estim : Inport  Port=2
  Bus Selector1 : BusSelector  OutputSignals=r
  Bus Selector5 : BusSelector  OutputSignals=yaw
  D_yaw : Gain  Gain=0.3*0.004
  Discrete-Time Integrator : DiscreteIntegrator  gainval=1  SampleTime=-1  ICPrevOutput=DiscIntNeverNeededParam  ICPrevScaledInput=DiscIntNeverNeededParam
  I_yaw : Gain  Gain=0.002  ParamDataTypeStr=single  OutDataTypeStr=single
  P_yaw : Gain  Gain=0.004  ParamDataTypeStr=single  OutDataTypeStr=single
  Saturation : Saturate  UpperLimit=pi/180*30  LowerLimit=-pi/180*30
  Sum1 : Sum  Inputs=|+-  OutDataTypeStr=single  AccumDataTypeStr=single  SaturateOnIntegerOverflow=on
  Sum2 : Sum  Inputs=++-
  tau_yaw : Outport  VectorParamsAs1DForOutWhenUnconnected=off
  wires:
  D_yaw/1 -> Sum2/3
  P_yaw/1 -> Sum2/1
  Bus Selector1/1 -> D_yaw/1  "<r>"
  Sum1/1 -> Saturation/1
  states_estim/1 -> Bus Selector1/1, Bus Selector5/1
  Bus Selector5/1 -> Sum1/2  "<yaw>"
  yaw_ref/1 -> Sum1/1
  Sum2/1 -> tau_yaw/1
  Discrete-Time Integrator/1 -> Sum2/2
  I_yaw/1 -> Discrete-Time Integrator/1
  Saturation/1 -> P_yaw/1, I_yaw/1

== system flightControlSystem/Control System/Controller/thrustsToMotorCommands ==
  thrusts_refin : Inport
  MotorDirections : Gain  Gain=[1 -1 1 -1]
  Saturation5 : Saturate  UpperLimit=Vehicle.Motor.maxLimit  LowerLimit=Vehicle.Motor.minLimit
  ThrustToMotorCommand : Gain  Gain=-Vehicle.Motor.thrustToMotorCommand
  motors_cmdout : Outport  VectorParamsAs1DForOutWhenUnconnected=off
  wires:
  Saturation5/1 -> MotorDirections/1
  MotorDirections/1 -> motors_cmdout/1
  ThrustToMotorCommand/1 -> Saturation5/1
  thrusts_refin/1 -> ThrustToMotorCommand/1

== system flightControlSystem/Control System/Crash Predictor Flags/Geofencing error ==
  Action Port : ActionPort  ActionPortLabel=if(u1 > 0)
  Constant : Constant  OutDataTypeStr=uint8
  Out1 : Outport  VectorParamsAs1DForOutWhenUnconnected=off
  wires:
  Constant/1 -> Out1/1

== system flightControlSystem/Control System/Crash Predictor Flags/No optical flow  ==
  Action Port : ActionPort  ActionPortLabel=elseif( u3> 0)
  Constant : Constant  Value=0  OutDataTypeStr=uint8
  Out1 : Outport  VectorParamsAs1DForOutWhenUnconnected=off
  wires:
  Constant/1 -> Out1/1

== system flightControlSystem/Control System/Crash Predictor Flags/Normal condition ==
  Action Port : ActionPort  ActionPortLabel=else
  Constant : Constant  Value=0  OutDataTypeStr=uint8
  Out1 : Outport  VectorParamsAs1DForOutWhenUnconnected=off
  wires:
  Constant/1 -> Out1/1

== system flightControlSystem/Control System/Crash Predictor Flags/Ultrasound improper ==
  Action Port : ActionPort  ActionPortLabel=elseif(u4>0)
  Constant : Constant  Value=0  OutDataTypeStr=uint8
  Out1 : Outport  VectorParamsAs1DForOutWhenUnconnected=off
  wires:
  Constant/1 -> Out1/1

== system flightControlSystem/Control System/Crash Predictor Flags/estimator//Optical flow error ==
  Action Port : ActionPort  ActionPortLabel=elseif(u2 > 0)
  Constant : Constant  Value=99  OutDataTypeStr=uint8
  Out1 : Outport  VectorParamsAs1DForOutWhenUnconnected=off
  wires:
  Constant/1 -> Out1/1

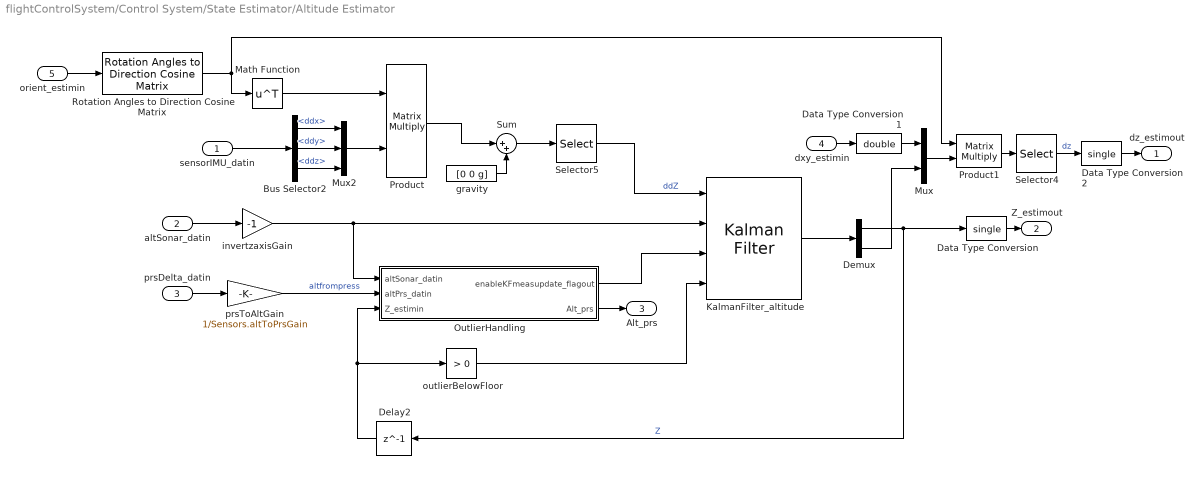
== system flightControlSystem/Control System/State Estimator/Altitude Estimator ==
  sensorIMU_datin : Inport
  altSonar_datin : Inport  Port=2
  prsDelta_datin : Inport  Port=3
  dxy_estimin : Inport  Port=4
  orient_estimin : Inport  Port=5
  Bus Selector2 : BusSelector  OutputSignals=ddx,ddy,ddz
  Data Type Conversion : DataTypeConversion  OutDataTypeStr=single  RndMeth=Floor
  Data Type Conversion1 : DataTypeConversion  OutDataTypeStr=double  RndMeth=Floor
  Data Type Conversion2 : DataTypeConversion  OutDataTypeStr=single  RndMeth=Floor
  Delay2 : Delay  DelayLength=1  InitialCondition=0
  Demux : Demux  Outputs=2
  KalmanFilter_altitude : ctrlSharedLib/Kalman Filter  TimeDomain=Discrete-Time  UseCurrentEstimator=on  ModelSource=Individual A, B, C, D matrices  ModelSourceVariable=sys  A=[1 Ts; 0 1]  B=[0;Ts]  C=[1 0]  D=[0]  NumberOfStates=2  NumberOfInputs=2  NumberOfOutputs=2  Ts=-1  InitialEstimateSource=Dialog  X0=[init.posNED(3) 0]  P0=10  UseK=off  UseGH=on  G=Estimator.alt.kf.G  TimeInvariantG=on  H=Estimator.alt.kf.H  TimeInvariantH=on  NumberOfProcessNoiseInputs=2  Q=Estimator.alt.kf.Q  TimeInvariantQ=on  R=Estimator.alt.kf.R  TimeInvariantR=on  N=Estimator.alt.kf.N  TimeInvariantN=on  AddInputPort=on  AddEnablePort=on  ExternalReset=Level hold  OutputEstimatedY=off  OutputP=off
  Math Function : Math  Operator=transpose  SignedPower=on
  Mux : Mux  Inputs=2
  Mux2 : Mux  Inputs=3
  OutlierHandling : Subsystem
  Product : Product  Multiplication=Matrix(*)
  Product1 : Product  Multiplication=Matrix(*)
  Rotation Angles to Direction Cosine Matrix : sharedtransform/Rotation Angles to Direction Cosine Matrix  rotationOrder=ZYX  aMode=aMode
  Selector4 : Selector  InputPortWidth=3  IndexOptions=Index vector (dialog)  Indices=[3]  OutputSizes=1
  Selector5 : Selector  InputPortWidth=3  IndexOptions=Index vector (dialog)  Indices=[3]  OutputSizes=1
  Sum : Sum  Inputs=|++
  gravity : Constant  Value=[0 0 g]
  invertzaxisGain : Gain  Gain=-1  ParamDataTypeStr=single  OutDataTypeStr=double
  outlierBelowFloor : simulink/Logic and Bit Operations/Compare To Constant  relop=>  const=0  OutDataTypeStr=boolean
  prsToAltGain : Gain  Gain=1/Sensors.altToPrsGain
  dz_estimout : Outport  VectorParamsAs1DForOutWhenUnconnected=off
  Z_estimout : Outport  Port=2  VectorParamsAs1DForOutWhenUnconnected=off
  Alt_prs : Outport  Port=3  VectorParamsAs1DForOutWhenUnconnected=off
  wires:
  Mux2/1 -> Product/2
  sensorIMU_datin/1 -> Bus Selector2/1
  Bus Selector2/3 -> Mux2/3  "<ddz>"
  Bus Selector2/2 -> Mux2/2  "<ddy>"
  Bus Selector2/1 -> Mux2/1  "<ddx>"
  Product1/1 -> Selector4/1
  dxy_estimin/1 -> Data Type Conversion1/1
  Delay2/1 -> OutlierHandling/3(Z_estimin), outlierBelowFloor/1
  prsToAltGain/1 -> OutlierHandling/2(altPrs_datin)  "altfrompress"
  prsDelta_datin/1 -> prsToAltGain/1
  outlierBelowFloor/1 -> KalmanFilter_altitude/4
  Demux/2 -> Mux/2
  Selector4/1 -> Data Type Conversion2/1  "dz"
  Demux/1 -> Data Type Conversion/1, Delay2/1  "Z"
  Selector5/1 -> KalmanFilter_altitude/1  "ddZ"
  Mux/1 -> Product1/2
  KalmanFilter_altitude/1 -> Demux/1
  Sum/1 -> Selector5/1
  gravity/1 -> Sum/2
  Product/1 -> Sum/1
  altSonar_datin/1 -> invertzaxisGain/1
  orient_estimin/1 -> Rotation Angles to Direction Cosine Matrix/1
  Data Type Conversion/1 -> Z_estimout/1
  Data Type Conversion1/1 -> Mux/1
  Math Function/1 -> Product/1
  invertzaxisGain/1 -> KalmanFilter_altitude/2, OutlierHandling/1(altSonar_datin)
  Data Type Conversion2/1 -> dz_estimout/1
  OutlierHandling/1(enableKFmeasupdate_flagout) -> KalmanFilter_altitude/3
  Rotation Angles to Direction Cosine Matrix/1 -> Math Function/1, Product1/1
  OutlierHandling/2(Alt_prs) -> Alt_prs/1
